simulink model "SIMULINK_convertidor_de_potencia"  (R2026a)
settings: Solver=ode45  StopTime=0.002  MaxStep=5e-7
InitFcn:
  | L = 0.002;
  | R = 10;
  | C = 10e-6;
  | Vin = 32;
settings Model: Creator=aizen  LastModifiedBy=aizen

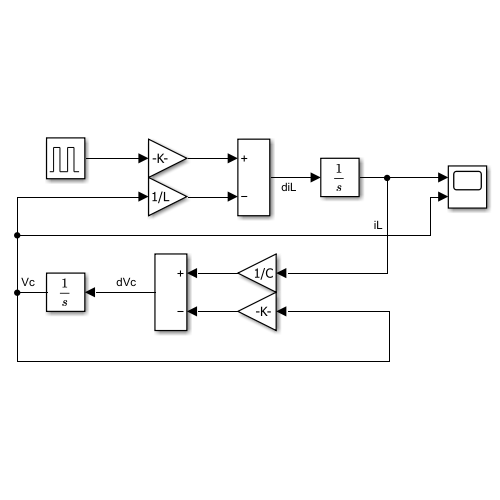
[thumbnail: Simulink's stored preview of the top-level diagram]
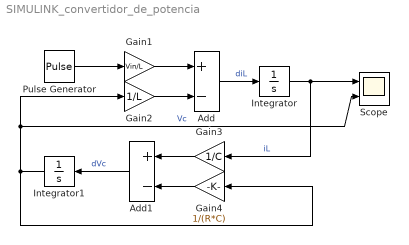
== system SIMULINK_convertidor_de_potencia ==
  Add : Sum  Inputs=+-
  Add1 : Sum  Inputs=+-
  Gain1 : Gain  Gain=Vin/L
  Gain2 : Gain  Gain=1/L
  Gain3 : Gain  Gain=1/C
  Gain4 : Gain  Gain=1/(R*C)
  Integrator : Integrator
  Integrator1 : Integrator
  Pulse Generator : DiscretePulseGenerator  PulseType=Time based  Period=10e-6  PulseWidth=40
  Scope : Scope  NumInputPorts=2
      settings: ActiveDisplayYMinimum=0.61737176745160482  ActiveDisplayYMaximum=1.5813713275185339
  wires:
  Pulse Generator/1 -> Gain1/1
  Gain1/1 -> Add/1
  Add/1 -> Integrator/1  "diL"
  Integrator/1 -> Gain3/1, Scope/1  "iL"
  Gain2/1 -> Add/2
  Integrator1/1 -> Scope/2, Gain2/1, Gain4/1  "Vc"
  Add1/1 -> Integrator1/1  "dVc"
  Gain3/1 -> Add1/1
  Gain4/1 -> Add1/2
